simulink model "lab6_task4_model1"  (R2024b)
settings: Solver=VariableStepAuto  StartTime=0.0  StopTime=10.0  RelTol=1e-3
libraries: simulink x1
settings Model: Creator=Beanie  LastModifiedBy=Beanie

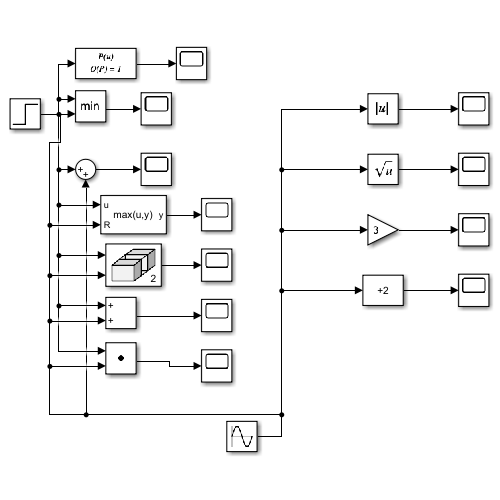
[thumbnail: Simulink's stored preview of the top-level diagram]
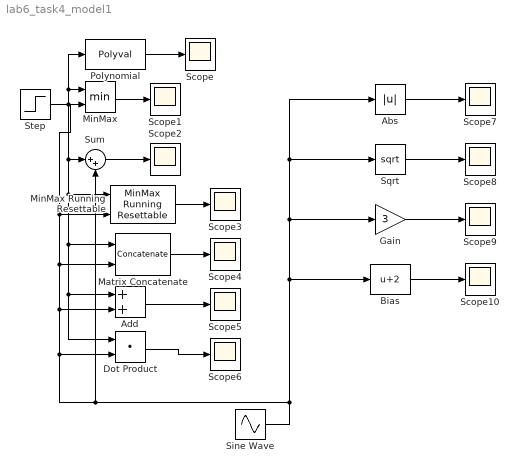
== system lab6_task4_model1 ==
  Abs : Abs  SaturateOnIntegerOverflow=off
  Add : Sum
  Bias : Bias  Bias=2  SaturateOnIntegerOverflow=off
  Dot Product : DotProduct  OutDataTypeStr=Inherit: Inherit via internal rule
  Gain : Gain  Gain=3
  Matrix Concatenate : Concatenate  Mode=Multidimensional array  ConcatenateDimension=2
  MinMax : MinMax  Inputs=2
  MinMax Running Resettable : simulink/Math Operations/MinMax Running Resettable  Function=max  vinit=0.0
  Polynomial : Polyval  Coefs=[1 0]
  Scope{,1..10} (11 alike) : Scope
  Sine Wave : Sin  Frequency=2*pi  SampleTime=0
  Sqrt : Sqrt
  Step : Step  SampleTime=0
  Sum : Sum  Inputs=|++
  wires:
  Step/1 -> Dot Product/1, Add/1, Matrix Concatenate/1, MinMax Running Resettable/1, Sum/1, Polynomial/1, MinMax/1
  Sine Wave/1 -> Abs/1, Sqrt/1, Gain/1, Bias/1, Add/2, Matrix Concatenate/2, MinMax/2, MinMax Running Resettable/2, Dot Product/2, Sum/2
  Bias/1 -> Scope10/1
  Gain/1 -> Scope9/1
  Sqrt/1 -> Scope8/1
  Abs/1 -> Scope7/1
  Dot Product/1 -> Scope6/1
  Add/1 -> Scope5/1
  Matrix Concatenate/1 -> Scope4/1
  MinMax Running Resettable/1 -> Scope3/1
  Sum/1 -> Scope2/1
  MinMax/1 -> Scope1/1
  Polynomial/1 -> Scope/1
